simulink model "EPS"  (R2024a)
settings: Solver=VariableStepAuto  StartTime=0.0  StopTime=10.0  RelTol=1e-3
undefined symbols (not defined in the file): assist_on, bm, bs, Jm, Js, K_l, Kd, Kts, N
settings Model: Creator=pc  LastModifiedBy=pc

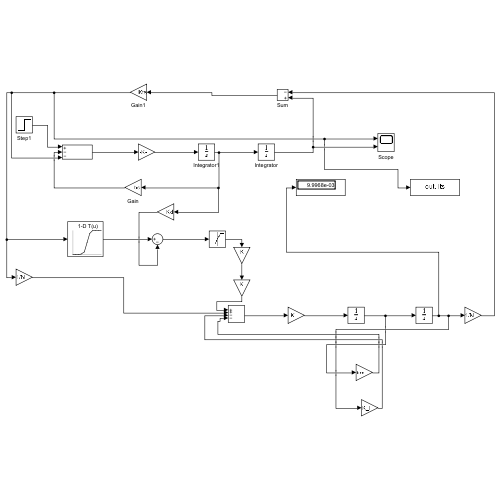
[thumbnail: Simulink's stored preview of the top-level diagram]
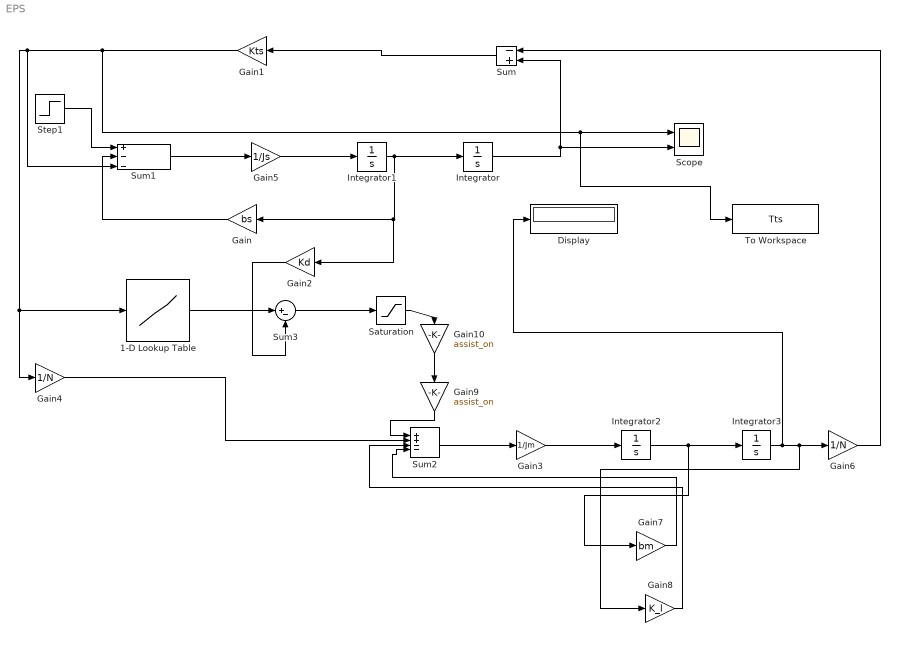
== system EPS ==
  1-D Lookup Table : Lookup_n-D  NumberOfTableDimensions=1  BreakpointsForDimension1=[-5:5]  Table=tanh([-5:5])  InternalRulePriority=Speed  RndMeth=Simplest
  Display : Display
      settings: Format=short_e
  Gain : Gain  Gain=bs
  Gain1 : Gain  Gain=Kts
  Gain10 : Gain  Gain=assist_on
  Gain2 : Gain  Gain=Kd
  Gain3 : Gain  Gain=1/Jm
  Gain4 : Gain  Gain=1/N
  Gain5 : Gain  Gain=1/Js
  Gain6 : Gain  Gain=1/N
  Gain7 : Gain  Gain=bm
  Gain8 : Gain  Gain=K_l
  Gain9 : Gain  Gain=assist_on
  Integrator{,1..3} (4 alike) : Integrator
  Saturation : Saturate  UpperLimit=5  LowerLimit=-5
  Scope : Scope  NumInputPorts=2
  Step1 : Step  After=3  SampleTime=0
  Sum : Sum  Inputs=-+
  Sum1 : Sum  Inputs=+--
  Sum2 : Sum  Inputs=++--
  Sum3 : Sum  Inputs=|+-
  To Workspace : ToWorkspace  VariableName=Tts  SaveFormat=Timeseries  SampleTime=-1
  wires:
  Integrator/1 -> Scope/2, Sum/2
  Sum1/1 -> Gain5/1
  Integrator1/1 -> Gain2/1, Gain/1, Integrator/1
  Sum/1 -> Gain1/1
  Gain/1 -> Sum1/2
  1-D Lookup Table/1 -> Sum3/1
  Sum3/1 -> Saturation/1
  Gain2/1 -> Sum3/2
  Gain4/1 -> Sum2/2
  Saturation/1 -> Gain10/1
  Sum2/1 -> Gain3/1
  Gain3/1 -> Integrator2/1
  Integrator2/1 -> Integrator3/1, Gain7/1
  Gain7/1 -> Sum2/4
  Gain8/1 -> Sum2/3
  Integrator3/1 -> Display/1, Gain8/1, Gain6/1
  Gain6/1 -> Sum/1
  Step1/1 -> Sum1/1
  Gain5/1 -> Integrator1/1
  Gain9/1 -> Sum2/1
  Gain10/1 -> Gain9/1
  Gain1/1 -> To Workspace/1, Scope/1, Sum1/3, Gain4/1, 1-D Lookup Table/1
